simulink library "ConverterLibrary"  (R2026a)
settings: Solver=VariableStepAuto
undefined symbols (not defined in the file or in its folder): DiscIntNeverNeededParam, dspblkCoreblockFVToolHelper, gcbh, gridInverter
libraries: fl_lib x240, nesl_utility x221, ee_lib x208, slpidlib x28, eeGeneralControl x12, simulink x9, eeTransforms x4, simulink_extras x1, eePowerMeasurement x1
(part 5 of 30)

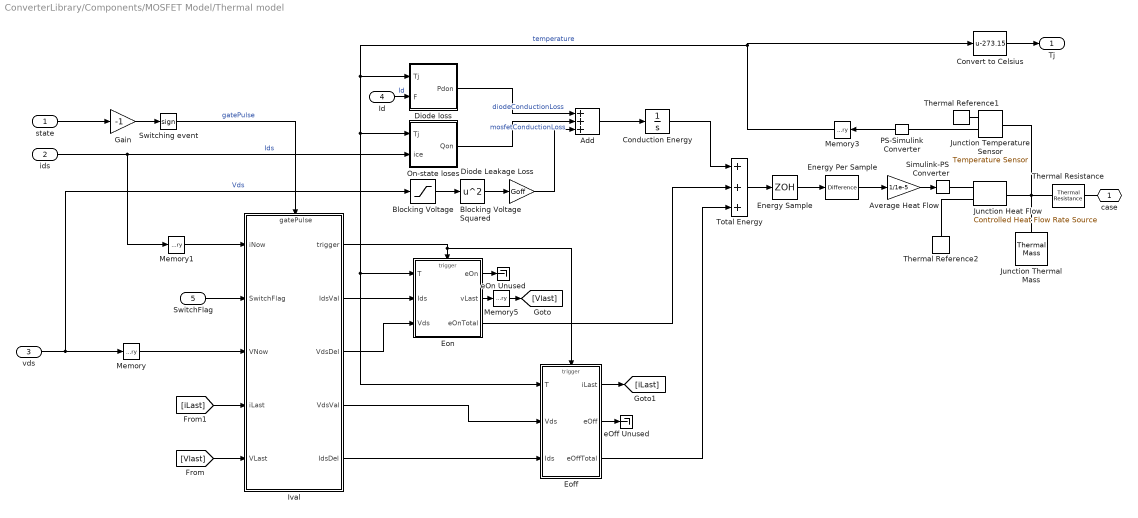
== system ConverterLibrary/Components/MOSFET Model/Thermal model ==
  state : Inport
  ids : Inport  Port=2
  vds : Inport  Port=3
  Id : Inport  Port=4
  SwitchFlag : Inport  Port=5
  Add : Sum  Inputs=+++
  Average Heat Flow : Gain  Gain=1/1e-5
  Blocking Voltage : Saturate  UpperLimit=inf  LowerLimit=0
  Blocking Voltage Squared : Math  Operator=square
  Conduction Energy : Integrator
  Convert to Celsius : Bias  Bias=-273.15  SaturateOnIntegerOverflow=off
  Diode Leakage Loss : Gain  Gain=Goff
  Diode loss : Subsystem
  Energy Per Sample : simulink/Discrete/Difference  ICPrevInput=0.0  OutMin=[]  OutMax=[]  OutDataType=fixdt(1, 16)  OutScaling=2^-10  DoSatur=off
  Energy Sample : ZeroOrderHold  SampleTime=1e-5
  Eoff : Subsystem
  Eon : Subsystem
  Gain : Gain  Gain=-1
  Ival : Subsystem
      settings: PortSchema="{\"entries\":[{\"content\":{\"sides\":[{\"content\":{\"connectorIds\":[\"In1\",\"In2\",\"In3\",\"In4\",\"In5\"]},\"type\":\"ConnectorPlacement.EquallySpacedRectSide\",\"uuid\":\"a553ebc5-b0a0-4a8e-bff0-a68d2801e087\"},{\"content\":{\"connectorIds\":[\"Out1\",\"Out2\",\"Out3\",\"Out4\",\"Out5\"],\"side\":\"RIGHT\"},\"type\":\"ConnectorPlacement.EquallySpacedRectSide\",\"uuid\":\"ac80ac7d-324c-4908-a07c-53a421efec51\"},{\"content\":{\"connectorIds\":[\"In6\"],\"side\":\"TOP\"},\"type\":\"ConnectorPlacement.EquallySpacedRectSide\",\"uuid\":\"7840bf98-6f1a-4afc-8020-e550163e4138\"}]},\"type\":\"ConnectorPlacement.EquallySpacedConnector\",\"uuid\":\"bf4a6777-16de-4536-9449-5f030ac27c09\"}],\"packageUris\":[\"http://schema.mathworks.com/mf0/Connector/R2020b\"],\"version\":\"1.0\"}"
  Junction Heat Flow : fl_lib/Thermal/Thermal Sources/Controlled Heat Flow Rate Source
  Junction Temperature Sensor : fl_lib/Thermal/Thermal Sensors/Temperature Sensor  temperature_measure=foundation.enum.MeasurementReference.difference
  Junction Thermal Mass : fl_lib/Thermal/Thermal Elements/Thermal Mass  mass_type=foundation.enum.constant_variable.constant  mass=thermal_mass kg  sp_heat=1 J/(K*kg)  mass_min=1e-6 kg  num_ports=foundation.enum.numPorts2.one  m_specify=off  m_priority=High  m=1 kg  m_nominal_specify=off  m_nominal_value=1  m_nominal_unit=kg  T_specify=on  T_priority=High  T=Tj0 K  T_nominal_specify=off  T_nominal_value=1  T_nominal_unit=K  Q_specify=off  Q_priority=None  Q=0 W  Q_nominal_specify=off  Q_nominal_value=1  Q_nominal_unit=W
  Memory : Memory  InitialCondition=Voff
  Memory1 : Memory
  Memory3 : Memory  InitialCondition=Tj0
  Memory5 : Memory
  On-state loses : Subsystem
  PS-Simulink Converter : nesl_utility/PS-Simulink Converter  PhysicalDomain=network_engine_domain  SubClassName=ps_output  LeftPortType=input  RightPortType=output  PseudoPeriodic=off  Frequencies=[]  VectorFormat=inherit  Unit=K  AffineConversion=off
  Simulink-PS Converter : nesl_utility/Simulink-PS Converter  PhysicalDomain=network_engine_domain  SubClassName=ps_input  LeftPortType=input  RightPortType=output  PseudoPeriodic=off  Frequencies=[]  NoiseDistribution=none  NoiseParameters=[]  Unit=W  AffineConversion=off  FilteringAndDerivatives=zero  SimscapeFilterOrder=1  InputFilterTimeConstant=0.001  UdotUserProvided=0
  Switching event : Signum
  Thermal Reference1 : fl_lib/Thermal/Thermal Elements/Thermal Reference
  Thermal Reference2 : fl_lib/Thermal/Thermal Elements/Thermal Reference
  Thermal Resistance : fl_lib/Thermal/Thermal Elements/Thermal Resistance  resistance=thermal_resistance K/W  T_specify=off  T_priority=None  T=0 K  T_nominal_specify=off  T_nominal_value=1  T_nominal_unit=K  Q_specify=off  Q_priority=None  Q=0 W  Q_nominal_specify=off  Q_nominal_value=1  Q_nominal_unit=W
  Total Energy : Sum  Inputs=+++
  eOff Unused : Terminator
  eOn Unused : Terminator
  case : PMIOPort  Side=Right
  Tj : Outport
  wires:
  Diode Leakage Loss/1 -> Add/3
  Blocking Voltage Squared/1 -> Diode Leakage Loss/1
  Blocking Voltage/1 -> Blocking Voltage Squared/1
  Diode loss/1(Pdon) -> Add/1  "diodeConductionLoss"
  Eoff/3(eOffTotal) -> Total Energy/3
  Eon/3(eOnTotal) -> Total Energy/2
  Conduction Energy/1 -> Total Energy/1
  Memory3/1 -> Eoff/1(T), Eon/1(T), On-state loses/1(Tj), Diode loss/1(Tj), Convert to Celsius/1  "temperature"
  Eoff/2(eOff) -> eOff Unused/1
  Eon/1(eOn) -> eOn Unused/1
  PS-Simulink Converter/1 -> Memory3/1
  Average Heat Flow/1 -> Simulink-PS Converter/1
  Energy Per Sample/1 -> Average Heat Flow/1
  Energy Sample/1 -> Energy Per Sample/1
  Total Energy/1 -> Energy Sample/1
  Add/1 -> Conduction Energy/1
  On-state loses/1(Qon) -> Add/2  "mosfetConductionLoss"
  Ival/5(IdsDel) -> Eoff/3(Ids)
  Ival/3(VdsDel) -> Eon/3(Vds)
  Ival/2(IdsVal) -> Eon/2(Ids)
  Memory/1 -> Ival/3(VNow)
  [Vlast] -> Ival/5(VLast)
  Ival/1(trigger) -> Eon/Trigger, Eoff/Trigger
  Ival/4(VdsVal) -> Eoff/2(Vds)
  [iLast] -> Ival/4(iLast)
  Gain/1 -> Switching event/1
  Eoff/1(iLast) -> [iLast]
  Memory5/1 -> [Vlast]
  SwitchFlag/1 -> Ival/2(SwitchFlag)
  Id/1 -> Diode loss/2(F)  "Id"
  vds/1 -> Blocking Voltage/1, Memory/1  "Vds"
  state/1 -> Gain/1
  Convert to Celsius/1 -> Tj/1
  Eon/2(vLast) -> Memory5/1
  Memory1/1 -> Ival/1(iNow)
  Switching event/1 -> Ival/6(gatePulse)  "gatePulse"
  ids/1 -> Memory1/1, On-state loses/2(ice)  "Ids"
  connections:
  Junction Temperature Sensor/RConn2 -- PS-Simulink Converter/LConn1
  Junction Temperature Sensor/RConn1 -- Thermal Reference1/LConn1
  Junction Heat Flow/RConn2 -- Thermal Reference2/LConn1
  Junction Heat Flow/RConn1 -- Simulink-PS Converter/RConn1
  Junction Temperature Sensor/LConn1 -- Thermal Resistance/RConn1 -- Junction Thermal Mass/LConn1 -- Junction Heat Flow/LConn1
  case/RConn1 -- Thermal Resistance/LConn1

== system ConverterLibrary/Controller/Inverter-Based Resources/Grid-Forming Converter Controller ==
  PrefPU : Inport
  QrefPU : Inport  Port=2
  IgabcPU : Inport  Port=3
  VgabcPU : Inport  Port=4
  Current Limiting : Subsystem
  Grid Voltage Reactive Power Support : Subsystem
  Measurement : Subsystem
      mask Display: image('$imagefile'); % Use "Edit Image" on toolstrip to change.
  Power Control : Subsystem
  Rate Transition3 : RateTransition
  VoltageCurrentControl : Subsystem
      settings: PortSchema="{\"entries\":[{\"content\":{\"sides\":[{\"content\":{\"connectorIds\":[\"In1\",\"In2\"]},\"type\":\"ConnectorPlacement.EquallySpacedRectSide\",\"uuid\":\"0bf15a12-7bc0-47e4-89bd-435769673763\"},{\"content\":{\"connectorIds\":[\"Out1\"],\"side\":\"RIGHT\"},\"type\":\"ConnectorPlacement.EquallySpacedRectSide\",\"uuid\":\"44a15d74-8878-4ec6-abe4-be0b1b609519\"},{\"content\":{\"connectorIds\":[\"In3\"],\"side\":\"TOP\"},\"type\":\"ConnectorPlacement.EquallySpacedRectSide\",\"uuid\":\"7a96781e-5638-4b2a-8101-d5785aae9f0f\"}]},\"type\":\"ConnectorPlacement.EquallySpacedConnector\",\"uuid\":\"4b3373ad-cf20-4175-894e-3bd1604dd0ce\"}],\"packageUris\":[\"http://schema.mathworks.com/mf0/Connector/R2020b\"],\"version\":\"1.0\"}"
  PmeasPU : Outport
  QmeasPU : Outport  Port=2
  FmeasHz : Outport  Port=3
  mabc : Outport  Port=4
  wires:
  Power Control/2(activeControl) -> VoltageCurrentControl/2(activeControl)
  Rate Transition3/1 -> Grid Voltage Reactive Power Support/1(measure), Power Control/1(measure), VoltageCurrentControl/3(measure), Current Limiting/1(measure)
  Measurement/4(FmeasHz) -> FmeasHz/1
  Grid Voltage Reactive Power Support/2(Qref) -> Power Control/3(Qref)
  Grid Voltage Reactive Power Support/1(Pref) -> Power Control/2(Pref)
  PrefPU/1 -> Grid Voltage Reactive Power Support/2(PrefInput)
  QrefPU/1 -> Grid Voltage Reactive Power Support/3(QrefInput)
  Current Limiting/1(currentLimiting) -> VoltageCurrentControl/1(currentLimiting)
  Power Control/1(reactiveControl) -> Current Limiting/2(reactiveControl)
  Power Control/3(angle) -> Measurement/3(Angle)
  Measurement/1(measure) -> Rate Transition3/1
  Measurement/3(QmeasPU) -> QmeasPU/1
  Measurement/2(PmeasPU) -> PmeasPU/1
  IgabcPU/1 -> Measurement/2(Igabc)
  VgabcPU/1 -> Measurement/1(Vgabcc)
  VoltageCurrentControl/1(mabc) -> mabc/1

== system ConverterLibrary/Controller/Non-Isolated DC-DC Converters/Non-Isolated DC-DC Controller ==
  Vref : Inport
  Vmeas : Inport  Port=2
  Imeas : Inport  Port=3
  Vin : Inport  Port=4
  Duty Feedforward : Subsystem
  Duty Rate Transition : RateTransition
  Duty Saturation : Saturate  UpperLimit=dutyMax  LowerLimit=dutyMin
  Loop Structure : Subsystem  Variant=on  VariantControlMode=label  LabelModeActiveChoice=DoubleLoop
  Output Mode : Subsystem  Variant=on  VariantControlMode=label  LabelModeActiveChoice=PWMSignal
  Per-Unit Scaling : Subsystem
  Sum : Sum  Inputs=|-+
  Sum1 : Sum  Inputs=|++
  Voltage Controller : Subsystem  Variant=on  VariantControlMode=label  LabelModeActiveChoice=PIContinuous
  G : Outport
  wires:
  Per-Unit Scaling/2(voltageReferencePu) -> Duty Feedforward/1(voltageReferencePu), Sum/2
  Output Mode/1(G) -> G/1
  Duty Rate Transition/1 -> Output Mode/1(duty)
  Duty Saturation/1 -> Duty Rate Transition/1
  Sum1/1 -> Duty Saturation/1
  Duty Feedforward/3(dutyFeedforward) -> Sum1/2
  Loop Structure/1(dutyTrim) -> Sum1/1
  Duty Feedforward/2(trimLowerLimit) -> Loop Structure/4(trimLowerLimit)
  Duty Feedforward/1(trimUpperLimit) -> Loop Structure/3(trimUpperLimit)
  Per-Unit Scaling/3(inductorCurrentPu) -> Loop Structure/2(inductorCurrentPu)
  Voltage Controller/1(vc) -> Loop Structure/1(voltageControllerOutput)
  Per-Unit Scaling/4(inputVoltagePuOut) -> Duty Feedforward/2(inputVoltagePuOut)
  Sum/1 -> Voltage Controller/1(error)
  Vin/1 -> Per-Unit Scaling/4(Vin)
  Imeas/1 -> Per-Unit Scaling/3(Imeas)
  Vmeas/1 -> Per-Unit Scaling/2(Vmeas)
  Vref/1 -> Per-Unit Scaling/1(Vref)
  Per-Unit Scaling/1(outputVoltagePu) -> Sum/1

== system ConverterLibrary/Controller/PWM Generators/CLLC PWM Generator ==
  fpu : Inport
  Isec : Inport  Port=2
  Frequency Limit : Saturate  UpperLimit=fpuMax  LowerLimit=fpuMin
  Primary Gate Signal : Subsystem
  Synchronous Rectifier : Subsystem
  G1 : Outport
  G2 : Outport  Port=2
  wires:
  fpu/1 -> Frequency Limit/1
  Frequency Limit/1 -> Primary Gate Signal/1(fpu), Synchronous Rectifier/2(fpu)
  Primary Gate Signal/2(gates) -> Synchronous Rectifier/1(primaryGates)
  Primary Gate Signal/1(G) -> G1/1
  Isec/1 -> Synchronous Rectifier/3(Isec)
  Synchronous Rectifier/1(Gs) -> G2/1

== system ConverterLibrary/Controller/PWM Generators/Complementary PWM Generator ==
  PWM : Inport
  Dead Time : Constant  Value=Tdead
  Delay Elapsed : Mux  Inputs=2
  Gate Level Offset : Bias  Bias=gateVoltageOff
  Gate Level Swing : Gain  Gain=gateVoltageOn - gateVoltageOff
  Gate Window : Logic
  Input Polarity : Mux  Inputs=2
  Input Threshold : RelationalOperator
  Inverted Input : Logic  Operator=NOT  Inputs=1
  Logic Threshold : Constant  Value=inputLogicThreshold
  Logic To Double : DataTypeConversion  OutDataTypeStr=double
  Ramp Floor : Constant  Value=0
  Ramp Mode : Subsystem  Variant=on  VariantControlMode=label  LabelModeActiveChoice=VariableStep
  Rate Offset : Bias  Bias=-1
  Rate Swing : Gain  Gain=2
  To Double : DataTypeConversion  OutDataTypeStr=double
  Turn Off Delay Elapsed : RelationalOperator  Operator=<=
  Turn On Delay Elapsed : RelationalOperator
  G : Outport
  wires:
  Gate Level Swing/1 -> Gate Level Offset/1
  PWM/1 -> Input Threshold/1
  Logic Threshold/1 -> Input Threshold/2
  Input Threshold/1 -> Logic To Double/1, Inverted Input/1, Input Polarity/1
  Inverted Input/1 -> Input Polarity/2
  Logic To Double/1 -> Rate Swing/1
  Rate Swing/1 -> Rate Offset/1
  Rate Offset/1 -> Ramp Mode/1(rate)
  Ramp Mode/1(S) -> Turn On Delay Elapsed/1, Turn Off Delay Elapsed/1
  Dead Time/1 -> Turn On Delay Elapsed/2
  Ramp Floor/1 -> Turn Off Delay Elapsed/2
  Turn On Delay Elapsed/1 -> Delay Elapsed/1
  Turn Off Delay Elapsed/1 -> Delay Elapsed/2
  Delay Elapsed/1 -> Gate Window/1
  Input Polarity/1 -> Gate Window/2
  Gate Window/1 -> To Double/1
  To Double/1 -> Gate Level Swing/1
  Gate Level Offset/1 -> G/1

== system ConverterLibrary/Controller/PWM Generators/DAB PWM Generator ==
  phaseShift : Inport
  pulseWidth : Inport  Port=2
  Dead Time : Constant  Value=Tdead
  Phase To Time : Gain  Gain=-1/(2*pi*Fsw)
  Primary Bridge Gate Map : Selector  InputPortWidth=2  IndexOptions=Index vector (dialog)  Indices=[1 2 2 1]  OutputSizes=1
  Primary Gate Level Offset : Bias  Bias=primaryGateVoltageOff
  Primary Gate Level Swing : Gain  Gain=primaryGateVoltageOn - primaryGateVoltageOff
  Primary Leg Gate Logic : Subsystem
  Pulse Time : Gain  Gain=1/Fsw
  Pulse Time Plus Dead Time : Bias  Bias=Tdead
  Pulse Width Limit : Saturate  UpperLimit=1 - Tdead*Fsw  LowerLimit=Tdead*Fsw
  Ramp Mode : Subsystem  Variant=on  VariantControlMode=label  LabelModeActiveChoice=VariableStep
  Secondary Bridge Gate Map : Selector  InputPortWidth=2  IndexOptions=Index vector (dialog)  Indices=[1 2 2 1]  OutputSizes=1
  Secondary Gate Level Offset : Bias  Bias=secondaryGateVoltageOff
  Secondary Gate Level Swing : Gain  Gain=secondaryGateVoltageOn - secondaryGateVoltageOff
  Secondary Leg Gate Logic : Subsystem
  Shifted Time : Sum
  Switching Period : Constant  Value=1/Fsw
  Turn Off Times : Mux  Inputs=2
  Turn On Times : Mux  Inputs=2
  Wrap To Period : Math  Operator=mod
  G1 : Outport
  G2 : Outport  Port=2
  wires:
  pulseWidth/1 -> Pulse Width Limit/1
  Pulse Width Limit/1 -> Pulse Time/1
  Pulse Time/1 -> Pulse Time Plus Dead Time/1, Turn Off Times/1
  Dead Time/1 -> Turn On Times/1
  Pulse Time Plus Dead Time/1 -> Turn On Times/2
  Switching Period/1 -> Turn Off Times/2, Ramp Mode/1(Tsw), Wrap To Period/2
  Primary Gate Level Swing/1 -> Primary Gate Level Offset/1
  Secondary Gate Level Swing/1 -> Secondary Gate Level Offset/1
  Turn On Times/1 -> Primary Leg Gate Logic/1(Ton), Secondary Leg Gate Logic/1(Ton)
  Turn Off Times/1 -> Primary Leg Gate Logic/2(Toff), Secondary Leg Gate Logic/2(Toff)
  Ramp Mode/1(S) -> Primary Leg Gate Logic/3(S), Shifted Time/1
  phaseShift/1 -> Phase To Time/1
  Phase To Time/1 -> Shifted Time/2
  Shifted Time/1 -> Wrap To Period/1
  Wrap To Period/1 -> Secondary Leg Gate Logic/3(S)
  Primary Leg Gate Logic/1(gates) -> Primary Bridge Gate Map/1
  Primary Bridge Gate Map/1 -> Primary Gate Level Swing/1
  Secondary Leg Gate Logic/1(gates) -> Secondary Bridge Gate Map/1
  Secondary Bridge Gate Map/1 -> Secondary Gate Level Swing/1
  Primary Gate Level Offset/1 -> G1/1
  Secondary Gate Level Offset/1 -> G2/1

== system ConverterLibrary/Controller/PWM Generators/Full Bridge PWM Generator ==
  duty : Inport
  Bridge Gate Map : Selector  InputPortWidth=2  IndexOptions=Index vector (dialog)  Indices=[1 2 2 1]  OutputSizes=1
  Dead Time : Constant  Value=Tdead
  Gate Level Offset : Bias  Bias=gateVoltageOff
  Gate Level Swing : Gain  Gain=gateVoltageOn - gateVoltageOff
  Leg Gate Logic : Subsystem
  Pulse Time : Gain  Gain=1/Fsw
  Pulse Time Plus Dead Time : Bias  Bias=Tdead
  Pulse Width Limit : Saturate  UpperLimit=1 - Tdead*Fsw  LowerLimit=Tdead*Fsw
  Ramp Mode : Subsystem  Variant=on  VariantControlMode=label  LabelModeActiveChoice=VariableStep
  Switching Period : Constant  Value=1/Fsw
  Turn Off Times : Mux  Inputs=2
  Turn On Times : Mux  Inputs=2
  G : Outport
  wires:
  duty/1 -> Pulse Width Limit/1
  Pulse Width Limit/1 -> Pulse Time/1
  Pulse Time/1 -> Pulse Time Plus Dead Time/1, Turn Off Times/1
  Dead Time/1 -> Turn On Times/1
  Pulse Time Plus Dead Time/1 -> Turn On Times/2
  Switching Period/1 -> Turn Off Times/2, Ramp Mode/1(Tsw)
  Gate Level Swing/1 -> Gate Level Offset/1
  Turn On Times/1 -> Leg Gate Logic/1(Ton)
  Turn Off Times/1 -> Leg Gate Logic/2(Toff)
  Ramp Mode/1(S) -> Leg Gate Logic/3(S)
  Leg Gate Logic/1(gates) -> Bridge Gate Map/1
  Bridge Gate Map/1 -> Gate Level Swing/1
  Gate Level Offset/1 -> G/1

== system ConverterLibrary/Controller/PWM Generators/Half Bridge PWM Generator ==
  duty : Inport
  Dead Time : Constant  Value=Tdead
  Gate Level Offset : Bias  Bias=gateVoltageOff
  Gate Level Swing : Gain  Gain=gateVoltageOn - gateVoltageOff
  Leg Gate Logic : Subsystem
  Pulse Time : Gain  Gain=1/Fsw
  Pulse Time Plus Dead Time : Bias  Bias=Tdead
  Pulse Width Limit : Saturate  UpperLimit=1 - Tdead*Fsw  LowerLimit=Tdead*Fsw
  Ramp Mode : Subsystem  Variant=on  VariantControlMode=label  LabelModeActiveChoice=VariableStep
  Switching Period : Constant  Value=1/Fsw
  Turn Off Times : Mux  Inputs=2
  Turn On Times : Mux  Inputs=2
  G : Outport
  wires:
  duty/1 -> Pulse Width Limit/1
  Pulse Width Limit/1 -> Pulse Time/1
  Pulse Time/1 -> Pulse Time Plus Dead Time/1, Turn Off Times/1
  Dead Time/1 -> Turn On Times/1
  Pulse Time Plus Dead Time/1 -> Turn On Times/2
  Switching Period/1 -> Turn Off Times/2, Ramp Mode/1(Tsw)
  Gate Level Swing/1 -> Gate Level Offset/1
  Turn On Times/1 -> Leg Gate Logic/1(Ton)
  Turn Off Times/1 -> Leg Gate Logic/2(Toff)
  Ramp Mode/1(S) -> Leg Gate Logic/3(S)
  Leg Gate Logic/1(gates) -> Gate Level Swing/1
  Gate Level Offset/1 -> G/1

== system ConverterLibrary/Controller/PWM Generators/LLC PWM Generator ==
  fpu : Inport
  Bridge Gate Map : Selector  InputPortWidth=2  IndexOptions=Index vector (dialog)  Indices=[1 2 2 1]  OutputSizes=1
  Dead Time : Constant  Value=Tdead
  Frequency Limit : Saturate  UpperLimit=fpuMax  LowerLimit=fpuMin
  Gate Level Offset : Bias  Bias=gateVoltageOff
  Gate Level Swing : Gain  Gain=gateVoltageOn - gateVoltageOff
  Hertz To Period : Math  Operator=reciprocal
  Leg Gate Logic : Subsystem
  Normalized To Hertz : Gain  Gain=Fbase
  Pulse Time : Gain  Gain=pulseWidth
  Pulse Time Plus Dead Time : Bias  Bias=Tdead
  Ramp Mode : Subsystem  Variant=on  VariantControlMode=label  LabelModeActiveChoice=VariableStep
  Turn Off Times : Mux  Inputs=2
  Turn On Times : Mux  Inputs=2
  G : Outport
  wires:
  Gate Level Swing/1 -> Gate Level Offset/1
  fpu/1 -> Frequency Limit/1
  Frequency Limit/1 -> Normalized To Hertz/1
  Normalized To Hertz/1 -> Hertz To Period/1
  Hertz To Period/1 -> Pulse Time/1, Turn Off Times/2, Ramp Mode/1(Tsw)
  Pulse Time/1 -> Pulse Time Plus Dead Time/1, Turn Off Times/1
  Dead Time/1 -> Turn On Times/1
  Pulse Time Plus Dead Time/1 -> Turn On Times/2
  Turn On Times/1 -> Leg Gate Logic/1(Ton)
  Turn Off Times/1 -> Leg Gate Logic/2(Toff)
  Ramp Mode/1(S) -> Leg Gate Logic/3(S)
  Leg Gate Logic/1(gates) -> Bridge Gate Map/1
  Bridge Gate Map/1 -> Gate Level Swing/1
  Gate Level Offset/1 -> G/1

== system ConverterLibrary/Controller/Power Factor Correction Converters/Boost PFC Controller ==
  Vref : Inport
  Vmeas : Inport  Port=2
  IL : Inport  Port=3
  Vac : Inport  Port=4
  Current Controller : Subsystem  Variant=on  VariantControlMode=label  LabelModeActiveChoice=PIContinuous
  Current Reference : Product
  Current Reference Limit : Saturate  UpperLimit=iRefPeakMaxPu  LowerLimit=0
  Duty Feedforward : Subsystem
  Duty Rate Transition : RateTransition
  Ierror : Sum  Inputs=|+-
  Output Mode : Subsystem  Variant=on  VariantControlMode=label  LabelModeActiveChoice=PWMSignal
  Per-Unit Scaling : Subsystem
  Pref : Constant  Value=PrefPu
  Sum : Sum  Inputs=|++
  Sum1 : Sum  Inputs=|++
  Verror : Sum  Inputs=|+-
  Voltage Controller : Subsystem  Variant=on  VariantControlMode=label  LabelModeActiveChoice=PIContinuous
  G : Outport
  wires:
  Duty Feedforward/2(trimLowerLimit) -> Current Controller/3(lo)
  [Iac] -> Ierror/2
  Per-Unit Scaling/4(absLineCurrentPuAC) -> [Iac]
  Output Mode/1(G) -> G/1
  Sum1/1 -> Duty Rate Transition/1
  Current Controller/1(vc) -> Sum1/1
  Duty Rate Transition/1 -> Output Mode/1(duty)
  Duty Feedforward/3(dutyFeedforward) -> Sum1/2
  Duty Feedforward/1(trimUpperLimit) -> Current Controller/2(up)
  Current Reference Limit/1 -> Ierror/1
  Current Reference/1 -> Current Reference Limit/1
  Sum/1 -> Current Reference/2
  Pref/1 -> Sum/2
  Voltage Controller/1(vc) -> Sum/1
  Verror/1 -> Voltage Controller/1(error)
  Per-Unit Scaling/5(absLineVoltagePuDC) -> Duty Feedforward/2(absLineVoltagePuDC)
  Ierror/1 -> Current Controller/1(error)
  Per-Unit Scaling/3(busVoltagePuDC) -> Verror/2, Duty Feedforward/1(busVoltagePuDC)
  Per-Unit Scaling/2(voltageReferencePuDC) -> Verror/1
  Vmeas/1 -> Per-Unit Scaling/3(Vmeas)
  Vref/1 -> Per-Unit Scaling/2(Vref)
  IL/1 -> Per-Unit Scaling/4(IL)
  Vac/1 -> Per-Unit Scaling/1(Vac)
  Per-Unit Scaling/1(absLineVoltagePuAC) -> Current Reference/1

== system ConverterLibrary/Controller/Power Factor Correction Converters/Interleaved Boost PFC Controller ==
  Vref : Inport
  Vmeas : Inport  Port=2
  IL1 : Inport  Port=3
  IL2 : Inport  Port=4
  Vac : Inport  Port=5
  Current Balance : Subsystem
  Current Controller : Subsystem  Variant=on  VariantControlMode=label  LabelModeActiveChoice=PIContinuous
  Current Reference : Product
  Current Reference Limit : Saturate  UpperLimit=iRefPeakMaxPu  LowerLimit=0
  Duty Feedforward : Subsystem
  Duty Rate Transition : RateTransition
  Duty Split : Subsystem
  Output Mode : Subsystem  Variant=on  VariantControlMode=label  LabelModeActiveChoice=PWMSignal
  Per-Unit Scaling : Subsystem
  Pref : Constant  Value=PrefPu
  Subtract : Sum  Inputs=-+
  Sum : Sum  Inputs=|++
  Sum1 : Sum  Inputs=|++
  Verror : Sum  Inputs=|+-
  Voltage Controller : Subsystem  Variant=on  VariantControlMode=label  LabelModeActiveChoice=PIContinuous
  G : Outport
  wires:
  Output Mode/1(G) -> G/1
  Duty Split/1(duty) -> Duty Rate Transition/1
  Sum1/1 -> Duty Split/1(dutyCommon)
  Duty Feedforward/2(trimLowerLimit) -> Current Controller/3(lo)
  Current Reference Limit/1 -> Subtract/2
  Current Reference/1 -> Current Reference Limit/1
  Sum/1 -> Current Reference/2
  Pref/1 -> Sum/2
  Voltage Controller/1(vc) -> Sum/1
  Duty Feedforward/3(dutyFeedforward) -> Sum1/2
  Current Balance/1(dutyTrim) -> Duty Split/2(dutyTrim)
  Per-Unit Scaling/7(leg2CurrentPuAC) -> Current Balance/2(leg2CurrentPuAC)
  Per-Unit Scaling/6(leg1CurrentPuAC) -> Current Balance/1(leg1CurrentPuAC)
  Per-Unit Scaling/5(absLineVoltagePuDC) -> Duty Feedforward/2(absLineVoltagePuDC)
  Per-Unit Scaling/1(absLineCurrentPuAC) -> Subtract/1
  Current Controller/1(vc) -> Sum1/1
  Duty Rate Transition/1 -> Output Mode/1(duty)
  Per-Unit Scaling/3(voltageReferencePuDC) -> Verror/1
  Per-Unit Scaling/2(absLineVoltagePuAC) -> Current Reference/1
  IL1/1 -> Per-Unit Scaling/4(IL1)
  Vmeas/1 -> Per-Unit Scaling/3(Vmeas)
  Vref/1 -> Per-Unit Scaling/2(Vref)
  Duty Feedforward/1(trimUpperLimit) -> Current Controller/2(up)
  Per-Unit Scaling/4(busVoltagePuDC) -> Verror/2, Duty Feedforward/1(busVoltagePuDC)
  Verror/1 -> Voltage Controller/1(error)
  Vac/1 -> Per-Unit Scaling/1(Vac)
  IL2/1 -> Per-Unit Scaling/5(IL2)
  Subtract/1 -> Current Controller/1(error)

== system ConverterLibrary/Controller/Power Factor Correction Converters/Totem-Pole Boost PFC Controller ==
  Vref : Inport
  Vmeas : Inport  Port=2
  Imeas : Inport  Port=3
  Vac : Inport  Port=4
  Current Controller : Subsystem  Variant=on  VariantControlMode=label  LabelModeActiveChoice=PIContinuous
  Current Reference : Product
  Current Reference Limit : Saturate  UpperLimit=iRefPeakMaxPu  LowerLimit=0
  Duty Feedforward : Subsystem
  Duty Rate Transition : RateTransition
  Gate Logic : Subsystem
  Ierror : Sum  Inputs=|+-
  Output Mode : Subsystem  Variant=on  VariantControlMode=label  LabelModeActiveChoice=PWMSignal
  Per-Unit Scaling : Subsystem
  Pref : Constant  Value=PrefPu
  Sum : Sum  Inputs=|++
  Sum1 : Sum  Inputs=|++
  Verror : Sum  Inputs=|+-
  Voltage Controller : Subsystem  Variant=on  VariantControlMode=label  LabelModeActiveChoice=PIContinuous
  G : Outport
  wires:
  Duty Feedforward/1(trimUpperLimit) -> Current Controller/2(up)
  Gate Logic/1(G) -> G/1
  Verror/1 -> Voltage Controller/1(error)
  Per-Unit Scaling/2(voltageReferencePuDC) -> Verror/1
  Duty Feedforward/2(trimLowerLimit) -> Current Controller/3(lo)
  Per-Unit Scaling/5(absLineVoltagePuDC) -> Duty Feedforward/2(absLineVoltagePuDC)
  Output Mode/1(G) -> Gate Logic/1(u)
  Duty Rate Transition/1 -> Output Mode/1(duty)
  Sum1/1 -> Duty Rate Transition/1
  Duty Feedforward/3(dutyFeedforward) -> Sum1/2
  Current Controller/1(vc) -> Sum1/1
  Ierror/1 -> Current Controller/1(error)
  Per-Unit Scaling/4(absLineCurrentPuAC) -> Ierror/2
  Current Reference Limit/1 -> Ierror/1
  Current Reference/1 -> Current Reference Limit/1
  Sum/1 -> Current Reference/2
  Pref/1 -> Sum/2
  Voltage Controller/1(vc) -> Sum/1
  Per-Unit Scaling/3(busVoltagePuDC) -> Duty Feedforward/1(busVoltagePuDC), Verror/2
  Per-Unit Scaling/6(lineVoltagePuAC) -> Gate Logic/2(Vac)
  Per-Unit Scaling/1(absLineVoltagePuAC) -> Current Reference/1
  Imeas/1 -> Per-Unit Scaling/4(Imeas)
  Vmeas/1 -> Per-Unit Scaling/3(Vmeas)
  Vref/1 -> Per-Unit Scaling/2(Vref)
  Vac/1 -> Per-Unit Scaling/1(Vac)

== system ConverterLibrary/Controller/Soft-Switching Converters/CLLC Controller ==
  Ref : Inport
  Ioutmeas : Inport  Port=2
  Iinmeas : Inport  Port=3
  VMeas : Inport  Port=4
  Iprimary : Inport  Port=5
  Isecondary : Inport  Port=6
  CCCV : Inport  Port=7
  mode : Inport  Port=8
  2P2Z Compensator : Subsystem  Variant=on  VariantControlMode=label  LabelModeActiveChoice=PIContinuous
  Gain : Gain  Gain=-1
  Gate Signal : Subsystem
  Switch : Switch  Criteria=u2 > Threshold  Threshold=0.5  SaturateOnIntegerOverflow=off  InputSameDT=off
  Unit Delay{,1..4} (5 alike) : UnitDelay  SampleTime=-1
  VCO : Subsystem  Variant=on  VariantControlMode=label  LabelModeActiveChoice=Constant
  Voltage Controller : Subsystem
      settings: PortSchema="{\"entries\":[{\"content\":{\"sides\":[{\"content\":{\"connectorIds\":[\"In1\",\"In2\",\"In3\"]},\"type\":\"ConnectorPlacement.EquallySpacedRectSide\",\"uuid\":\"f0fd2bba-62ea-41fa-9e2d-20e9baca433d\"},{\"content\":{\"connectorIds\":[\"Out1\"],\"side\":\"RIGHT\"},\"type\":\"ConnectorPlacement.EquallySpacedRectSide\",\"uuid\":\"b07713f3-6482-4c49-813d-98ee62fb3af9\"},{\"content\":{\"connectorIds\":[\"In4\"],\"side\":\"TOP\"},\"type\":\"ConnectorPlacement.EquallySpacedRectSide\",\"uuid\":\"b625d4be-27a7-4d9d-bcc3-22a88b5ba553\"}]},\"type\":\"ConnectorPlacement.EquallySpacedConnector\",\"uuid\":\"a8d6e586-eb25-49bc-834f-41a4855fcd05\"}],\"packageUris\":[\"http://schema.mathworks.com/mf0/Connector/R2020b\"],\"version\":\"1.0\"}"
  Gp : Outport
  Gs : Outport  Port=2
  wires:
  Unit Delay4/1 -> Gate Signal/4(Iprimary)
  Unit Delay3/1 -> Gate Signal/3(Isecondary)
  2P2Z Compensator/1(vc) -> VCO/1(vc)
  Gain/1 -> Switch/3
  Unit Delay2/1 -> Gain/1
  Switch/1 -> Voltage Controller/3(Imeas)
  Unit Delay1/1 -> Switch/1
  Iinmeas/1 -> Unit Delay2/1
  Ref/1 -> Voltage Controller/1(Ref)  "ref"
  Ioutmeas/1 -> Unit Delay1/1
  CCCV/1 -> Voltage Controller/4(CCCV)  "CCCV"
  Voltage Controller/1(Ierr) -> 2P2Z Compensator/1(error)
  Iprimary/1 -> Unit Delay4/1  "Vout"
  Isecondary/1 -> Unit Delay3/1  "Vout"
  mode/1 -> Switch/2, Gate Signal/2(mode)  "Vout"
  Gate Signal/2(G2) -> Gs/1
  VMeas/1 -> Unit Delay/1  "Vout"
  VCO/1(f) -> Gate Signal/1(f)
  Gate Signal/1(G1) -> Gp/1
  Unit Delay/1 -> Voltage Controller/2(Vmeas)

== system ConverterLibrary/Controller/Soft-Switching Converters/DAB Controller (SPS) ==
  Ref : Inport
  Vmeas : Inport  Port=2
  Imeas : Inport  Port=3
  CCCV : Inport  Port=4
  CC-CV Control : Subsystem
  Output Mode : Subsystem  Variant=on  VariantControlMode=label  LabelModeActiveChoice=PWMSignal
  G1 : Outport
  G2 : Outport  Port=2
  wires:
  CC-CV Control/1(phaseShift) -> Output Mode/1(phaseShift)
  Output Mode/1(G1) -> G1/1
  Output Mode/2(G2) -> G2/1
  Ref/1 -> CC-CV Control/1(Ref)
  Vmeas/1 -> CC-CV Control/2(Vmeas)
  Imeas/1 -> CC-CV Control/3(Imeas)
  CCCV/1 -> CC-CV Control/4(CCCV)

== system ConverterLibrary/Controller/Soft-Switching Converters/LLC Voltage Controller ==
  Ref : Inport
  Meas : Inport  Port=2
  2P2Z Compensator : Subsystem  Variant=on  VariantControlMode=label  LabelModeActiveChoice=SCompensator
  LLC PWM Generator : Subsystem
  LLCerror : Sum  Inputs=|-+
  Unit Delay : UnitDelay  SampleTime=-1
  VCO : Subsystem  Variant=on  VariantControlMode=label  LabelModeActiveChoice=Constant
  G : Outport
  wires:
  LLC PWM Generator/1(G) -> G/1  "llcGates"
  VCO/1(f) -> LLC PWM Generator/1(fpu)
  Meas/1 -> Unit Delay/1  "Vout"
  2P2Z Compensator/1(vc) -> VCO/1(vc)
  Unit Delay/1 -> LLCerror/2
  LLCerror/1 -> 2P2Z Compensator/1(error)
  Ref/1 -> LLCerror/1  "Vref"

== system ConverterLibrary/Power Converter Plant/Non-Isolated DC-DC Converters/Non-Isolated DC-DC Converter ==
  G : Inport
  NonIsolatedDCDCVariant : Subsystem  Variant=on  VariantControlMode=label  LabelModeActiveChoice=SynchronousBoost
  Vin+ : PMIOPort  Side=Left
  Vin- : PMIOPort  Port=2  Side=Left
  Vout+ : PMIOPort  Port=3  Side=Right
  Vout- : PMIOPort  Port=4  Side=Right
  meas : Outport
  wires:
  G/1 -> NonIsolatedDCDCVariant/1(G)
  NonIsolatedDCDCVariant/1(meas) -> meas/1
  connections:
  Vin+/RConn1 -- NonIsolatedDCDCVariant/LConn1
  Vin-/RConn1 -- NonIsolatedDCDCVariant/LConn2
  NonIsolatedDCDCVariant/RConn1 -- Vout+/RConn1
  NonIsolatedDCDCVariant/RConn2 -- Vout-/RConn1

== system ConverterLibrary/Power Converter Plant/Power Factor Correction Converters/Boost PFC Converter ==
  G : Inport
  BoostPFCVariant : Subsystem  Variant=on  VariantControlMode=label  LabelModeActiveChoice=SimplifiedModel
  P : PMIOPort  Side=Left
  N : PMIOPort  Port=2  Side=Left
  + : PMIOPort  Port=3  Side=Right
  - : PMIOPort  Port=4  Side=Right
  meas : Outport
  wires:
  G/1 -> BoostPFCVariant/1(G)
  BoostPFCVariant/1(meas) -> meas/1
  connections:
  P/RConn1 -- BoostPFCVariant/LConn1
  N/RConn1 -- BoostPFCVariant/LConn2
  BoostPFCVariant/RConn1 -- +/RConn1
  BoostPFCVariant/RConn2 -- -/RConn1

== system ConverterLibrary/Power Converter Plant/Power Factor Correction Converters/Interleaved Boost PFC Converter ==
  G : Inport
  InterleavedBoostPFCVariant : Subsystem  Variant=on  VariantControlMode=label  LabelModeActiveChoice=SimplifiedModel
  P : PMIOPort  Side=Left
  N : PMIOPort  Port=2  Side=Left
  + : PMIOPort  Port=3  Side=Right
  - : PMIOPort  Port=4  Side=Right
  meas : Outport
  wires:
  G/1 -> InterleavedBoostPFCVariant/1(G)
  InterleavedBoostPFCVariant/1(meas) -> meas/1
  connections:
  P/RConn1 -- InterleavedBoostPFCVariant/LConn1
  N/RConn1 -- InterleavedBoostPFCVariant/LConn2
  InterleavedBoostPFCVariant/RConn1 -- +/RConn1
  InterleavedBoostPFCVariant/RConn2 -- -/RConn1

== system ConverterLibrary/Power Converter Plant/Power Factor Correction Converters/Totem-Pole Boost PFC Converter ==
  G : Inport
  TotemPoleBoostPFCVariant : Subsystem  Variant=on  VariantControlMode=label  LabelModeActiveChoice=SimplifiedModel
  P : PMIOPort  Side=Left
  N : PMIOPort  Port=2  Side=Left
  + : PMIOPort  Port=3  Side=Right
  - : PMIOPort  Port=4  Side=Right
  meas : Outport
  wires:
  TotemPoleBoostPFCVariant/1(meas) -> meas/1
  G/1 -> TotemPoleBoostPFCVariant/1(G)
  connections:
  TotemPoleBoostPFCVariant/RConn2 -- -/RConn1
  TotemPoleBoostPFCVariant/RConn1 -- +/RConn1
  N/RConn1 -- TotemPoleBoostPFCVariant/LConn2
  P/RConn1 -- TotemPoleBoostPFCVariant/LConn1

== system ConverterLibrary/Power Converter Plant/Soft-Switching Converters/CLLC Converter ==
  Gpri : Inport
  Gsec : Inport  Port=2
  CLLCConverterVariant : Subsystem  Variant=on  VariantControlMode=label  LabelModeActiveChoice=SimplifiedModel
  P1 : PMIOPort  Side=Left
  N1 : PMIOPort  Port=2  Side=Left
  P2 : PMIOPort  Port=3  Side=Right
  N2 : PMIOPort  Port=4  Side=Right
  Meas : Outport
  wires:
  Gpri/1 -> CLLCConverterVariant/1(Gpri)
  Gsec/1 -> CLLCConverterVariant/2(Gsec)
  CLLCConverterVariant/1(Meas) -> Meas/1
  connections:
  CLLCConverterVariant/LConn1 -- P1/RConn1
  CLLCConverterVariant/LConn2 -- N1/RConn1
  CLLCConverterVariant/RConn1 -- P2/RConn1
  CLLCConverterVariant/RConn2 -- N2/RConn1

== system ConverterLibrary/Power Converter Plant/Soft-Switching Converters/DAB Converter ==
  Gp : Inport
  Gs : Inport  Port=2
  DABConverterVariant : Subsystem  Variant=on  VariantControlMode=label  LabelModeActiveChoice=DetailedModel
      settings: PortSchema="{\"entries\":[{\"content\":{\"sides\":[{\"content\":{\"connectorIds\":[\"In1\",\"LConn1\",\"LConn2\"]},\"type\":\"ConnectorPlacement.EquallySpacedRectSide\",\"uuid\":\"6f245ee7-ecea-433e-8ace-55b7238b8bbd\"},{\"content\":{\"connectorIds\":[\"In2\",\"Out1\",\"RConn1\",\"RConn2\"],\"side\":\"RIGHT\"},\"type\":\"ConnectorPlacement.EquallySpacedRectSide\",\"uuid\":\"af7f8c88-8cd1-4285-8228-b98ea57f06ae\"},{\"content\":{\"side\":\"TOP\"},\"type\":\"ConnectorPlacement.EquallySpacedRectSide\",\"uuid\":\"820d378e-11b2-4797-9989-1ab18f65f7f5\"}]},\"type\":\"ConnectorPlacement.EquallySpacedConnector\",\"uuid\":\"ae0f71da-cdc3-4120-89e7-21ff59b441bf\"}],\"packageUris\":[\"http://schema.mathworks.com/mf0/Connector/R2020b\"],\"version\":\"1.0\"}"
  P1 : PMIOPort  Side=Left
  N1 : PMIOPort  Port=2  Side=Left
  P2 : PMIOPort  Port=3  Side=Right
  N2 : PMIOPort  Port=4  Side=Right
  meas : Outport
  wires:
  DABConverterVariant/1(meas) -> meas/1
  Gs/1 -> DABConverterVariant/2(Gs)
  Gp/1 -> DABConverterVariant/1(Gp)
  connections:
  P1/RConn1 -- DABConverterVariant/LConn1
  N1/RConn1 -- DABConverterVariant/LConn2
  DABConverterVariant/RConn1 -- P2/RConn1
  DABConverterVariant/RConn2 -- N2/RConn1

== system ConverterLibrary/Power Converter Plant/Soft-Switching Converters/LLC Converter ==
  G : Inport
  Bus Creator : BusCreator  Inputs=3
  LLC Primary Inverter and Resonant Tank : Subsystem  Variant=on  VariantControlMode=label  LabelModeActiveChoice=DetailedModel
  Rectifier : Subsystem
      settings: PortSchema="{\"entries\":[{\"content\":{\"sides\":[{\"content\":{\"connectorIds\":[\"LConn1\",\"LConn2\",\"LConn3\"]},\"type\":\"ConnectorPlacement.EquallySpacedRectSide\",\"uuid\":\"4786b3cc-2245-4c72-a50b-9c63e4ad3d8a\"},{\"content\":{\"connectorIds\":[\"RConn1\",\"RConn2\"],\"side\":\"RIGHT\"},\"type\":\"ConnectorPlacement.EquallySpacedRectSide\",\"uuid\":\"250a01d0-bf95-4e01-bf69-d866bcf3b7bd\"},{\"content\":{\"connectorIds\":[\"Out1\"],\"side\":\"TOP\"},\"type\":\"ConnectorPlacement.EquallySpacedRectSide\",\"uuid\":\"52730d18-084b-4644-8b2a-b54c84fa88ec\"}]},\"type\":\"ConnectorPlacement.EquallySpacedConnector\",\"uuid\":\"d24cae2a-f132-4f5a-ac35-d7440d7a99e9\"}],\"packageUris\":[\"http://schema.mathworks.com/mf0/Connector/R2020b\"],\"version\":\"1.0\"}"
  + : PMIOPort  Side=Left
  +1 : PMIOPort  Port=2  Side=Right
  - : PMIOPort  Port=3  Side=Left
  -1 : PMIOPort  Port=4  Side=Right
  meas : Outport
  wires:
  Bus Creator/1 -> meas/1
  LLC Primary Inverter and Resonant Tank/2(measTank) -> Bus Creator/2
  LLC Primary Inverter and Resonant Tank/1(measInv) -> Bus Creator/1
  G/1 -> LLC Primary Inverter and Resonant Tank/1(G)
  Rectifier/1(meas) -> Bus Creator/3  "Rectifier"
  connections:
  LLC Primary Inverter and Resonant Tank/RConn3 -- Rectifier/LConn3
  LLC Primary Inverter and Resonant Tank/RConn2 -- Rectifier/LConn2
  LLC Primary Inverter and Resonant Tank/RConn1 -- Rectifier/LConn1
  LLC Primary Inverter and Resonant Tank/LConn2 -- -/RConn1
  LLC Primary Inverter and Resonant Tank/LConn1 -- +/RConn1
  -1/RConn1 -- Rectifier/RConn2
  +1/RConn1 -- Rectifier/RConn1

== system ConverterLibrary/Components/Diode Model/Thermal model/Diode loss ==
  Tj : Inport
  F : Inport  Port=2
  I-V : Lookup_n-D  BreakpointsForDimension1=Tj_diode  BreakpointsForDimension2=If_data  Table=Vf_data  InternalRulePriority=Speed  RndMeth=Simplest
      settings: InputPortMap=u0,u1
  On-state losses : Product
  Saturation : Saturate  UpperLimit=inf  LowerLimit=0
  Pdon : Outport
  wires:
  F/1 -> I-V/2, On-state losses/2
  I-V/1 -> On-state losses/1
  On-state losses/1 -> Saturation/1
  Tj/1 -> I-V/1
  Saturation/1 -> Pdon/1

== system ConverterLibrary/Components/Diode Model/Thermal model/Reverse recovery ==
  T : Inport
  If : Inport  Port=2
  Vr : Inport  Port=3
  Trigger : TriggerPort  VariantControl=(inherit)  PortDimensions=1
  Energy Total : Sum
  Erec : Lookup_n-D  BreakpointsForDimension1=Tj_rec  BreakpointsForDimension2=If_rec_data  BreakpointsForDimension3=[5, 7]  Table=Erec_data  InternalRulePriority=Speed  RndMeth=Simplest
      settings: InputPortMap=u0,u1
  Previous Total : UnitDelay  SampleTime=-1
  Product : Product
  Voltage scaling : Gain  Gain=1/Vrec_ref
  eRec : Outport
  eRecTotal : Outport  Port=2
  wires:
  T/1 -> Erec/1
  If/1 -> Erec/2
  Erec/1 -> Product/1
  Vr/1 -> Voltage scaling/1
  Voltage scaling/1 -> Product/2
  Product/1 -> eRec/1, Energy Total/1
  Energy Total/1 -> eRecTotal/1, Previous Total/1
  Previous Total/1 -> Energy Total/2

== system ConverterLibrary/Components/IGBT Model/Antiparallel Diode/ExternalDiode ==
  Open Circuit N : fl_lib/Electrical/Electrical Elements/Open Circuit  v_specify=off  v_priority=None  v=0 V  v_nominal_specify=off  v_nominal_value=1  v_nominal_unit=V
  Open Circuit P : fl_lib/Electrical/Electrical Elements/Open Circuit  v_specify=off  v_priority=None  v=0 V  v_nominal_specify=off  v_nominal_value=1  v_nominal_unit=V
  Zero Diode Current : Constant  Value=0
  P : PMIOPort  Side=Left
  N : PMIOPort  Port=2  Side=Left
  Id : Outport
  wires:
  Zero Diode Current/1 -> Id/1
  connections:
  P/RConn1 -- Open Circuit P/LConn1
  N/RConn1 -- Open Circuit N/LConn1

== system ConverterLibrary/Components/IGBT Model/Antiparallel Diode/InbuiltDiode ==
  Diode : fl_lib/Electrical/Electrical Elements/Diode  Vf=diodeVf V  Ron=diodeRon Ohm  Goff=diodeGoff 1/Ohm  i_specify=off  i_priority=None  i=0 A  i_nominal_specify=off  i_nominal_value=1  i_nominal_unit=A  v_specify=off  v_priority=None  v=0 V  v_nominal_specify=off  v_nominal_value=1  v_nominal_unit=V
  Probe : SimscapeProbe  BoundBlock=5850  Variables="{\"i\":{\"Probing\":\"ON\"}}"
  P : PMIOPort  Side=Left
  N : PMIOPort  Port=2  Side=Left
  Id : Outport
  wires:
  Probe/1 -> Id/1
  connections:
  N/RConn1 -- Diode/LConn1
  P/RConn1 -- Diode/RConn1

== system ConverterLibrary/Components/IGBT Model/Thermal model/Diode loss ==
  Tj : Inport
  F : Inport  Port=2
  I-V : Lookup_n-D  BreakpointsForDimension1=Tj_diode  BreakpointsForDimension2=If_data  Table=Vf_data  InternalRulePriority=Speed  RndMeth=Simplest
      settings: InputPortMap=u0,u1
  On-state losses : Product
  Saturation : Saturate  UpperLimit=inf  LowerLimit=0
  Pdon : Outport
  wires:
  F/1 -> I-V/2, On-state losses/2
  I-V/1 -> On-state losses/1
  On-state losses/1 -> Saturation/1
  Tj/1 -> I-V/1
  Saturation/1 -> Pdon/1

== system ConverterLibrary/Components/IGBT Model/Thermal model/Eoff ==
  T : Inport
  Vds : Inport  Port=2
  iCE : Inport  Port=3
  Trigger : TriggerPort  TriggerType=falling  VariantControl=(inherit)  ZeroCross=off  InitialTriggerSignalState=zero  PortDimensions=1
  1/Voff : Gain  Gain=1/Voff
  Energy Total : Sum
  Eoff : Lookup_n-D  BreakpointsForDimension1=Tj_loss  BreakpointsForDimension2=Iout_data_loss  Table=Eoff_data  InternalRulePriority=Speed  RndMeth=Simplest
      settings: InputPortMap=u0,u1
  Previous Total : UnitDelay  SampleTime=-1
  Product : Product
  iLast : Outport
  eOff : Outport  Port=2
  eOffTotal : Outport  Port=3
  wires:
  T/1 -> Eoff/1
  iCE/1 -> iLast/1, Eoff/2
  1/Voff/1 -> Product/2
  Eoff/1 -> Product/1
  Product/1 -> eOff/1, Energy Total/1
  Vds/1 -> 1/Voff/1
  Energy Total/1 -> eOffTotal/1, Previous Total/1
  Previous Total/1 -> Energy Total/2

== system ConverterLibrary/Components/IGBT Model/Thermal model/Eon ==
  T : Inport
  Ids : Inport  Port=2
  vCE : Inport  Port=3
  Trigger : TriggerPort  VariantControl=(inherit)  ZeroCross=off  InitialTriggerSignalState=zero  PortDimensions=1
  1/Voff : Gain  Gain=1/Voff
  Energy Total : Sum
  Eon : Lookup_n-D  BreakpointsForDimension1=Tj_loss  BreakpointsForDimension2=Iout_data_loss  Table=Eon_data  InternalRulePriority=Speed  RndMeth=Simplest
      settings: InputPortMap=u0,u1
  Previous Total : UnitDelay  SampleTime=-1
  Product : Product
  eOn : Outport
  vLast : Outport  Port=2
  eOnTotal : Outport  Port=3
  wires:
  T/1 -> Eon/1
  vCE/1 -> 1/Voff/1, vLast/1
  Eon/1 -> Product/1
  1/Voff/1 -> Product/2
  Product/1 -> eOn/1, Energy Total/1
  Ids/1 -> Eon/2
  Energy Total/1 -> eOnTotal/1, Previous Total/1
  Previous Total/1 -> Energy Total/2

== system ConverterLibrary/Components/IGBT Model/Thermal model/Ival ==
  iNow : Inport
  SwitchFlag : Inport  Port=2
  VNow : Inport  Port=3
  iLast : Inport  Port=4
  VLast : Inport  Port=5
  gatePulse : Inport  Port=6
  Current Delay : Memory
  Gate Pulse Delay : Memory
  Switch{,1..4} (5 alike) : Switch  Criteria=u2 > Threshold  Threshold=0.5  SaturateOnIntegerOverflow=off  InputSameDT=off
  Voltage Delay : Memory
  trigger : Outport
  IdsVal : Outport  Port=2
  VdsDel : Outport  Port=3
  VdsVal : Outport  Port=4
  IdsDel : Outport  Port=5
  wires:
  iLast/1 -> Switch/3
  SwitchFlag/1 -> Switch3/2, Switch4/2, Switch2/2, Switch1/2, Switch/2
  iNow/1 -> Switch4/3, Current Delay/1, Switch/1  "inow"
  Switch/1 -> IdsVal/1
  Gate Pulse Delay/1 -> Switch1/1
  gatePulse/1 -> Switch1/3, Gate Pulse Delay/1
  Switch1/1 -> trigger/1
  VNow/1 -> Switch3/3, Voltage Delay/1, Switch2/1  "inow"
  Switch2/1 -> VdsVal/1
  VLast/1 -> Switch2/3
  Switch3/1 -> VdsDel/1
  Switch4/1 -> IdsDel/1
  Voltage Delay/1 -> Switch3/1
  Current Delay/1 -> Switch4/1

== system ConverterLibrary/Components/IGBT Model/Thermal model/On-state loses ==
  Tj : Inport
  ice : Inport  Port=2
  I-V : Lookup_n-D  BreakpointsForDimension1=Tj  BreakpointsForDimension2=Iout_data  Table=Von_data  InternalRulePriority=Speed  RndMeth=Simplest
      settings: InputPortMap=u0,u1
  On-state losses : Product
  Saturation : Saturate  UpperLimit=inf  LowerLimit=0
  Qon : Outport
  wires:
  ice/1 -> I-V/2, On-state losses/2
  I-V/1 -> On-state losses/1
  On-state losses/1 -> Saturation/1
  Tj/1 -> I-V/1
  Saturation/1 -> Qon/1

== system ConverterLibrary/Components/MOSFET Model/Thermal model/Diode loss ==
  Tj : Inport
  F : Inport  Port=2
  I-V : Lookup_n-D  BreakpointsForDimension1=Tj_diode  BreakpointsForDimension2=If_data  Table=Vf_data  InternalRulePriority=Speed  RndMeth=Simplest
      settings: InputPortMap=u0,u1
  On-state losses : Product
  Saturation : Saturate  UpperLimit=inf  LowerLimit=0
  Pdon : Outport
  wires:
  Saturation/1 -> Pdon/1
  Tj/1 -> I-V/1
  On-state losses/1 -> Saturation/1
  I-V/1 -> On-state losses/1
  F/1 -> On-state losses/2, I-V/2

== system ConverterLibrary/Components/MOSFET Model/Thermal model/Eoff ==
  T : Inport
  Vds : Inport  Port=2
  Ids : Inport  Port=3
  Trigger : TriggerPort  TriggerType=falling  VariantControl=(inherit)  ZeroCross=off  InitialTriggerSignalState=zero  PortDimensions=1
  1/Voff : Gain  Gain=1/Voff
  Energy Total : Sum
  Eoff : Lookup_n-D  BreakpointsForDimension1=Tj_loss  BreakpointsForDimension2=Iout_data_loss  Table=Eoff_data  InternalRulePriority=Speed  RndMeth=Simplest
      settings: InputPortMap=u0,u1
  Previous Total : UnitDelay  SampleTime=-1
  Product : Product
  iLast : Outport
  eOff : Outport  Port=2
  eOffTotal : Outport  Port=3
  wires:
  Previous Total/1 -> Energy Total/2
  Energy Total/1 -> Previous Total/1, eOffTotal/1
  Vds/1 -> 1/Voff/1
  Product/1 -> Energy Total/1, eOff/1
  Eoff/1 -> Product/1
  1/Voff/1 -> Product/2
  Ids/1 -> Eoff/2, iLast/1
  T/1 -> Eoff/1

== system ConverterLibrary/Components/MOSFET Model/Thermal model/Eon ==
  T : Inport
  Ids : Inport  Port=2
  Vds : Inport  Port=3
  Trigger : TriggerPort  VariantControl=(inherit)  ZeroCross=off  InitialTriggerSignalState=zero  PortDimensions=1
  1/Voff : Gain  Gain=1/Voff
  Energy Total : Sum
  Eon : Lookup_n-D  BreakpointsForDimension1=Tj_loss  BreakpointsForDimension2=Iout_data_loss  Table=Eon_data  InternalRulePriority=Speed  RndMeth=Simplest
      settings: InputPortMap=u0,u1
  Previous Total : UnitDelay  SampleTime=-1
  Product : Product
  eOn : Outport
  vLast : Outport  Port=2
  eOnTotal : Outport  Port=3
  wires:
  Previous Total/1 -> Energy Total/2
  Energy Total/1 -> Previous Total/1, eOnTotal/1
  Ids/1 -> Eon/2
  Product/1 -> Energy Total/1, eOn/1
  1/Voff/1 -> Product/2
  Eon/1 -> Product/1
  Vds/1 -> 1/Voff/1, vLast/1
  T/1 -> Eon/1

== system ConverterLibrary/Components/MOSFET Model/Thermal model/Ival ==
  iNow : Inport
  SwitchFlag : Inport  Port=2
  VNow : Inport  Port=3
  iLast : Inport  Port=4
  VLast : Inport  Port=5
  gatePulse : Inport  Port=6
  Current Delay : Memory
  Gate Pulse Delay : Memory
  Switch{,1..4} (5 alike) : Switch  Criteria=u2 > Threshold  Threshold=0.5  SaturateOnIntegerOverflow=off  InputSameDT=off
  Voltage Delay : Memory
  trigger : Outport
  IdsVal : Outport  Port=2
  VdsDel : Outport  Port=3
  VdsVal : Outport  Port=4
  IdsDel : Outport  Port=5
  wires:
  Current Delay/1 -> Switch4/1
  Voltage Delay/1 -> Switch3/1
  Switch4/1 -> IdsDel/1
  Switch3/1 -> VdsDel/1
  VLast/1 -> Switch2/3
  Switch2/1 -> VdsVal/1
  VNow/1 -> Switch2/1, Voltage Delay/1, Switch3/3  "inow"
  Switch1/1 -> trigger/1
  gatePulse/1 -> Gate Pulse Delay/1, Switch1/3
  Gate Pulse Delay/1 -> Switch1/1
  Switch/1 -> IdsVal/1
  iNow/1 -> Switch/1, Current Delay/1, Switch4/3  "inow"
  SwitchFlag/1 -> Switch/2, Switch1/2, Switch2/2, Switch4/2, Switch3/2
  iLast/1 -> Switch/3

== system ConverterLibrary/Components/MOSFET Model/Thermal model/On-state loses ==
  Tj : Inport
  ice : Inport  Port=2
  I-V : Lookup_n-D  BreakpointsForDimension1=Tj  BreakpointsForDimension2=Iout_data  Table=Von_data  InternalRulePriority=Speed  RndMeth=Simplest
      settings: InputPortMap=u0,u1
  On-state losses : Product
  Saturation : Saturate  UpperLimit=inf  LowerLimit=0
  Qon : Outport
  wires:
  Saturation/1 -> Qon/1
  Tj/1 -> I-V/1
  On-state losses/1 -> Saturation/1
  I-V/1 -> On-state losses/1
  ice/1 -> On-state losses/2, I-V/2

== system ConverterLibrary/Controller/Inverter-Based Resources/Grid-Forming Converter Controller/Current Limiting ==
  In Bus Element : Inport  PortName=measure  Element=Igd
  In Bus Element1 : Inport  PortName=measure  Element=Igq
  In Bus Element2 : Inport  Port=2  PortName=reactiveControl  Element=Vmd
  In Bus Element4 : Inport  Port=2  PortName=reactiveControl  Element=Vmq
  CurrentLimitingMethod : Subsystem  Variant=on  VariantControlMode=label  VariantControl=Choice  LabelModeActiveChoice=virimp
  Subtract : Sum  Inputs=+-
  Subtract1 : Sum  Inputs=-+
  Out Bus Element : Outport  PortName=currentLimiting  Element=Vmd
  Out Bus Element1 : Outport  PortName=currentLimiting  Element=Vmq
  Out Bus Element2 : Outport  PortName=currentLimiting  Element=Idmax
  Out Bus Element3 : Outport  PortName=currentLimiting  Element=Iqmax
  wires:
  CurrentLimitingMethod/4(Iqmax) -> Out Bus Element3/1
  CurrentLimitingMethod/3(Idmax) -> Out Bus Element2/1
  CurrentLimitingMethod/2(delVq) -> Subtract1/1
  CurrentLimitingMethod/1(delVd) -> Subtract/2
  In Bus Element/1 -> CurrentLimitingMethod/1(Igd)  "Q"
  Subtract1/1 -> Out Bus Element1/1
  Subtract/1 -> Out Bus Element/1
  In Bus Element4/1 -> Subtract1/2
  In Bus Element1/1 -> CurrentLimitingMethod/2(Igq)
  In Bus Element2/1 -> Subtract/1

== system ConverterLibrary/Controller/Inverter-Based Resources/Grid-Forming Converter Controller/Grid Voltage Reactive Power Support ==
  In Bus Element1 : Inport  PortName=measure  Element=Vgd
  In Bus Element3 : Inport  PortName=measure  Element=Vgq
  In Bus Element2 : Inport  PortName=measure  Element=Igd
  In Bus Element4 : Inport  PortName=measure  Element=Igq
  PrefInput : Inport  Port=2
  QrefInput : Inport  Port=3
  Modifying Active Power Reference : Subsystem
  Modifying Reactive Power Reference : Subsystem
  Rate Transition{,1..5} (6 alike) : RateTransition
  Pref : Outport
  Qref : Outport  Port=2
  wires:
  Rate Transition/1 -> Modifying Active Power Reference/2(Vd), Modifying Reactive Power Reference/1(Vgd)
  Rate Transition5/1 -> Qref/1
  Rate Transition4/1 -> Pref/1
  Rate Transition1/1 -> Modifying Reactive Power Reference/4(Pref)
  Rate Transition3/1 -> Modifying Reactive Power Reference/3(Qref)
  Rate Transition2/1 -> Modifying Reactive Power Reference/2(Vgq)
  Modifying Active Power Reference/1(Pref) -> Rate Transition1/1
  In Bus Element1/1 -> Rate Transition/1
  Modifying Reactive Power Reference/2(QrefNew) -> Rate Transition5/1
  Modifying Reactive Power Reference/1(PrefNew) -> Rate Transition4/1
  QrefInput/1 -> Rate Transition3/1
  In Bus Element3/1 -> Rate Transition2/1
  In Bus Element4/1 -> Modifying Active Power Reference/4(Igq)
  In Bus Element2/1 -> Modifying Active Power Reference/3(Igd)
  PrefInput/1 -> Modifying Active Power Reference/1(PrefInput)
